simulink model "SITRA_S2_test"  (R2026a)
settings: Solver=FixedStepDiscrete  StartTime=0  StopTime=600  FixedStep=1
model workspace (MAT data in the model file):
  T = 600
  cycleLength = 63
  dt = 1
  maxGreen = 30
  minGreen = 12
  normalDemand = [0.1 0.07 0.05]
  surgeDemand = [0.3 0.07 0.05]
  surgeEnd = 400
  surgeStart = 200
  yellowTime = 3
Description:
  | S1 architecture for the SITRA traffic-management and power-electronics implementation roadmap.
  | 
  | Reference traffic network: HopeCollege, Kalapatti, Airport -> SITRA -> Goldwins.
  | Frozen Part 8 MPC is the supervisory reference controller.
  | S1 contains architecture only; detailed dynamics are implemented later.
  | 
  | Simulation parameters:
  | dt = 1.0 s
  | T = 600.0 s
  | Cycle = 63.0 s
  | Yellow/Clearance = 3.0 s
  | Minimum green = 12.0 s
  | Maximum green = 30.0 s
  | Normal demand = [0.10 0.07 0.05] veh/s
  | Surge demand = [0.30 0.07 0.05] veh/s
  | Surge interval = 200.0 to 400.0 s
settings Model: Creator=Sreedev  LastModifiedBy=Sreedev

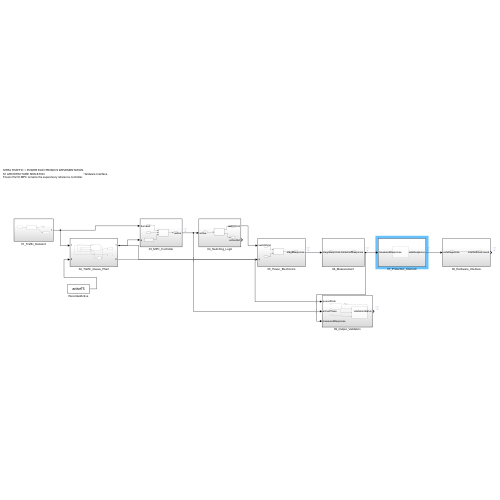
[thumbnail: Simulink's stored preview of the top-level diagram]
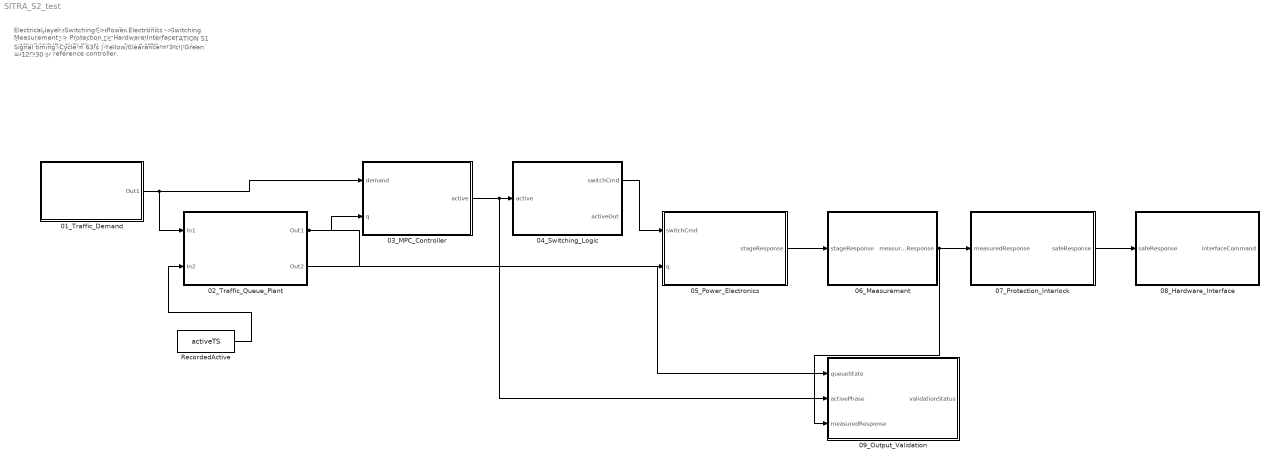
== system SITRA_S2_test ==
  note: SITRA TRAFFIC + POWER ELECTRONICS IMPLEMENTATION
      | S1 ARCHITECTURE SKELETON
      | Frozen Part 8 MPC remains the supervisory reference controller.
  note: Traffic layer:
      | Demand -> Queue Plant -> MPC -> Switching
  note: Electrical layer:
      | Switching -> Power Electronics -> Measurement -> Protection -> Hardware Interface
  note: Signal timing:
      | Cycle = 63 s | Yellow/Clearance = 3 s | Green = 12...30 s
  01_Traffic_Demand : Subsystem
  02_Traffic_Queue_Plant : Subsystem
  03_MPC_Controller : Subsystem
  04_Switching_Logic : Subsystem
  05_Power_Electronics : Subsystem
  06_Measurement : Subsystem
  07_Protection_Interlock : Subsystem
  08_Hardware_Interface : Subsystem
  09_Output_Validation : Subsystem
  RecordedActive : FromWorkspace  VariableName=activeTS  SampleTime=1  Interpolate=off  OutputAfterFinalValue=Holding final value
  wires:
  01_Traffic_Demand/1(Out1) -> 02_Traffic_Queue_Plant/1(In1), 03_MPC_Controller/1(demand)
  02_Traffic_Queue_Plant/1(Out1) -> 03_MPC_Controller/2(q), 05_Power_Electronics/2(q)
  03_MPC_Controller/1(active) -> 04_Switching_Logic/1(active), 09_Output_Validation/2(activePhase)
  05_Power_Electronics/1(stageResponse) -> 06_Measurement/1(stageResponse)
  06_Measurement/1(measuredResponse) -> 07_Protection_Interlock/1(measuredResponse), 09_Output_Validation/3(measuredResponse)
  07_Protection_Interlock/1(safeResponse) -> 08_Hardware_Interface/1(safeResponse)
  02_Traffic_Queue_Plant/2(Out2) -> 09_Output_Validation/1(queueState)
  RecordedActive/1 -> 02_Traffic_Queue_Plant/2(In2)
  04_Switching_Logic/1(switchCmd) -> 05_Power_Electronics/1(switchCmd)

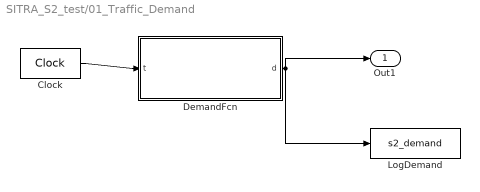
== system SITRA_S2_test/01_Traffic_Demand ==
  Clock : DigitalClock
  DemandFcn : MATLAB Function  TreatAsAtomicUnit=on
  LogDemand : ToWorkspace  VariableName=s2_demand  SampleTime=1
  Out1 : Outport
  wires:
  Clock/1 -> DemandFcn/1(t)
  DemandFcn/1(d) -> Out1/1, LogDemand/1

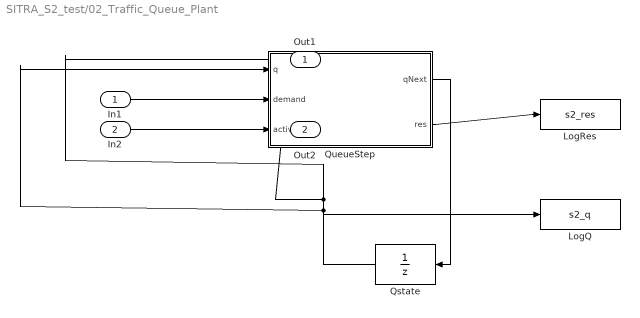
== system SITRA_S2_test/02_Traffic_Queue_Plant ==
  In1 : Inport
  In2 : Inport  Port=2
  LogQ : ToWorkspace  VariableName=s2_q  SampleTime=1
  LogRes : ToWorkspace  VariableName=s2_res  SampleTime=1
  Qstate : UnitDelay  InitialCondition=zeros(4,1)
  QueueStep : MATLAB Function  TreatAsAtomicUnit=on
  Out1 : Outport
  Out2 : Outport  Port=2
  wires:
  Qstate/1 -> Out1/1, Out2/1, QueueStep/1(q), LogQ/1
  In1/1 -> QueueStep/2(demand)
  In2/1 -> QueueStep/3(active)
  QueueStep/1(qNext) -> Qstate/1
  QueueStep/2(res) -> LogRes/1

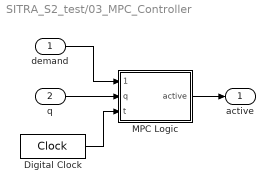
== system SITRA_S2_test/03_MPC_Controller ==
  demand : Inport
  q : Inport  Port=2
  Digital Clock : DigitalClock
  MPC Logic : MATLAB Function  TreatAsAtomicUnit=on
  active : Outport
  wires:
  demand/1 -> MPC Logic/1(demand)
  q/1 -> MPC Logic/2(q)
  Digital Clock/1 -> MPC Logic/3(t)
  MPC Logic/1(active) -> active/1

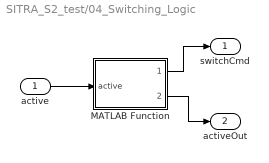
== system SITRA_S2_test/04_Switching_Logic ==
  active : Inport
  MATLAB Function : MATLAB Function  TreatAsAtomicUnit=on
  switchCmd : Outport
  activeOut : Outport  Port=2
  wires:
  MATLAB Function/1(switchCmd) -> switchCmd/1
  MATLAB Function/2(activeOut) -> activeOut/1
  active/1 -> MATLAB Function/1(active)

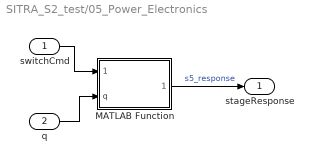
== system SITRA_S2_test/05_Power_Electronics ==
  switchCmd : Inport
  q : Inport  Port=2
  MATLAB Function : MATLAB Function  TreatAsAtomicUnit=on
  stageResponse : Outport
  wires:
  switchCmd/1 -> MATLAB Function/1(switchCmd)
  q/1 -> MATLAB Function/2(q)
  MATLAB Function/1(stageResponse) -> stageResponse/1  "s5_response"

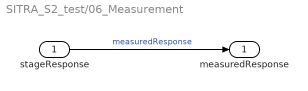
== system SITRA_S2_test/06_Measurement ==
  stageResponse : Inport
  measuredResponse : Outport
  wires:
  stageResponse/1 -> measuredResponse/1  "measuredResponse"

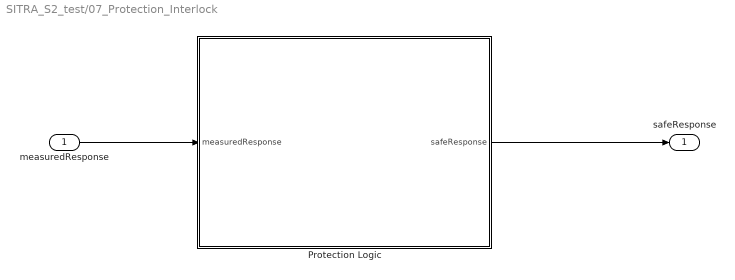
== system SITRA_S2_test/07_Protection_Interlock ==
  measuredResponse : Inport
  Protection Logic : MATLAB Function  TreatAsAtomicUnit=on
  safeResponse : Outport
  wires:
  measuredResponse/1 -> Protection Logic/1(measuredResponse)
  Protection Logic/1(safeResponse) -> safeResponse/1

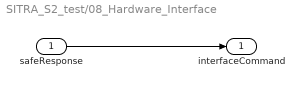
== system SITRA_S2_test/08_Hardware_Interface ==
  safeResponse : Inport
  interfaceCommand : Outport
  wires:
  safeResponse/1 -> interfaceCommand/1

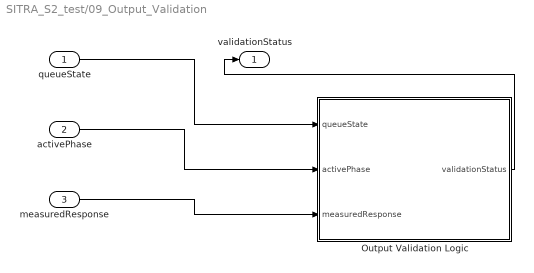
== system SITRA_S2_test/09_Output_Validation ==
  queueState : Inport
  activePhase : Inport  Port=2
  measuredResponse : Inport  Port=3
  Output Validation Logic : MATLAB Function  TreatAsAtomicUnit=on
  validationStatus : Outport
  wires:
  queueState/1 -> Output Validation Logic/1(queueState)
  activePhase/1 -> Output Validation Logic/2(activePhase)
  measuredResponse/1 -> Output Validation Logic/3(measuredResponse)
  Output Validation Logic/1(validationStatus) -> validationStatus/1

== matlab function SITRA_S2_test/01_Traffic_Demand/DemandFcn ==
  data: t input; d output
function d = demandProfile(t)
% Normal / surge demand [B1 B2 B3] veh/s (matches Part 8)
normalD = [0.10 0.07 0.05];
surgeD  = [0.30 0.07 0.05];
if t >= 200 && t < 400
    d = surgeD;
else
    d = normalD;
end
end

== matlab function SITRA_S2_test/02_Traffic_Queue_Plant/QueueStep ==
  data: q input; qNext output; demand input; active input; res output
function [qNext, res] = queueStep(q, demand, active)
% Four-branch traffic queue plant

% Ensure column vectors
q = q(:);
demand = demand(:);

% Branch capacities
cap = [0.65; 0.35; 0.25; 0.45];

dt = 1;

% Arrivals and departures
arr = [demand; 0];
dep = zeros(4,1);

a = round(active);

if a >= 1 && a <= 3
    dep(a) = min(cap(a), q(a)/dt);
    arr(4) = dep(a);
end

dep(4) = min(cap(4), q(4)/dt);

% Queue update
qNext = max(zeros(4,1), q + dt*(arr-dep));

% Conservation residual
res = arr-dep-(qNext-q)/dt;

end

== matlab function SITRA_S2_test/03_MPC_Controller/MPC Logic ==
  data: demand input; active output; q input; t input
function active = fcn(demand, q, t)
% SITRA MPC Traffic Signal Controller
% Inputs:
% demand = traffic demand [B1 B2 B3]
% q      = queue lengths [B1 B2 B3 B4]
% t      = simulation time

% Ensure row vectors
demand = reshape(demand,1,3);
q = reshape(q,1,4);

% Controller parameters
n = 3;
yellow = 3;
cycleLength = 63;
minGreen = 12;
maxGreen = 30;

totalGreen = cycleLength - n*yellow;

% Initial green allocation
base = minGreen*ones(1,n);
remaining = totalGreen - sum(base);

% Predictive priority score
score = max(q(1:n),0) + 10*max(demand,0);
score(2:3) = score(2:3) + 0.25;

% Allocate remaining green time
greenTimes = base;

for s = 1:round(remaining)

    room = maxGreen - greenTimes;
    [m,idx] = max(score .* (room > 1e-12));

    if m <= 0
        break;
    end

    greenTimes(idx) = greenTimes(idx) + 1;
    score(idx) = score(idx)*0.985 + 1e-12;

end

% Correct rounding mismatch
diffGreen = totalGreen - sum(greenTimes);

while abs(diffGreen) > 1e-12

    if diffGreen > 0
        room = maxGreen-greenTimes;
        [mx,idx] = max(room);

        if mx <= 0
            break;
        end

        add = min(diffGreen,mx);
        greenTimes(idx) = greenTimes(idx)+add;

    else
        room = greenTimes-minGreen;
        [mx,idx] = max(room);

        if mx <= 0
            break;
        end

        sub = min(-diffGreen,mx);
        greenTimes(idx) = greenTimes(idx)-sub;
    end

    diffGreen = totalGreen-sum(greenTimes);

end

% Determine active traffic branch
tau = mod(t,cycleLength);
current = 0;
active = 0;

for p = 1:n

    gEnd = current + greenTimes(p);
    yEnd = gEnd + yellow;

    if tau >= current && tau < gEnd
        active = p;
        return;

    elseif tau >= gEnd && tau < yEnd
        active = 0;
        return;
    end

    current = yEnd;

end

end

== matlab function SITRA_S2_test/04_Switching_Logic/MATLAB Function ==
  data: active input; switchCmd output; activeOut output
function [switchCmd, activeOut] = fcn(active)
% SITRA Switching Logic

% Initialize all switches OFF
switchCmd = zeros(1,3);

% Validate and decode MPC output
a = round(active);

if a >= 1 && a <= 3
    switchCmd(a) = 1;
    activeOut = a;
else
    activeOut = 0;
end

end

== matlab function SITRA_S2_test/05_Power_Electronics/MATLAB Function ==
  data: switchCmd input; stageResponse output; q input
function stageResponse = fcn(switchCmd, q)
% SITRA S5 - Behavioural Power Electronics Model
% No physical component ratings assumed.

% Convert inputs to row vectors
switchCmd = reshape(switchCmd,1,3);
q = reshape(q,1,4);

% Initialize output
stageResponse = 0;

% Validate switching commands
validBinary = all((switchCmd == 0) | (switchCmd == 1));

mutualExclusion = sum(switchCmd) <= 1;

validQueue = all(q >= 0);

if validBinary && mutualExclusion && validQueue

    % Behavioural load response of selected branch
    stageResponse = sum(switchCmd .* q(1:3));

else

    % Invalid switching state: stage disabled
    stageResponse = 0;

end

end

== matlab function SITRA_S2_test/07_Protection_Interlock/Protection Logic ==
  data: measuredResponse input; safeResponse output
function safeResponse = fcn(measuredResponse)

safeResponse = 0;

if isreal(measuredResponse) && ...
   ~isnan(measuredResponse) && ...
   ~isinf(measuredResponse) && ...
   measuredResponse >= 0

    safeResponse = measuredResponse;
end

end

== matlab function SITRA_S2_test/09_Output_Validation/Output Validation Logic ==
  data: queueState input; validationStatus output; activePhase input; measuredResponse input
function validationStatus = fcn(queueState, activePhase, measuredResponse)
queueState = queueState(:);
queueValid = all(isfinite(queueState) & queueState >= 0);
activeValid = isfinite(activePhase) && activePhase >= 0 && ...
activePhase <= 3 && activePhase == round(activePhase);
measurementValid = isfinite(measuredResponse) && measuredResponse >= 0;
validationStatus = double(queueValid && activeValid && measurementValid);
end
